simulink model "normal"  (R2023a)
settings: Solver=VariableStepAuto  StartTime=0.0  StopTime=0.2  RelTol=1e-3
libraries: spsMosfetLib x4, spsOnDelayLib x4, spsCurrentMeasurementLib x1, spsDCVoltageSourceLib x1, spsSeriesRLCLoadLib x1, spsTriangleGeneratorLib x1, spsVoltageMeasurementLib x1, sps_lib x1
settings Model: Creator=student  LastModifiedBy=student

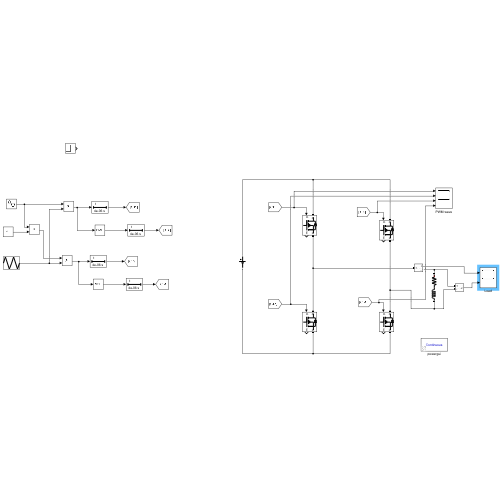
[thumbnail: Simulink's stored preview of the top-level diagram]
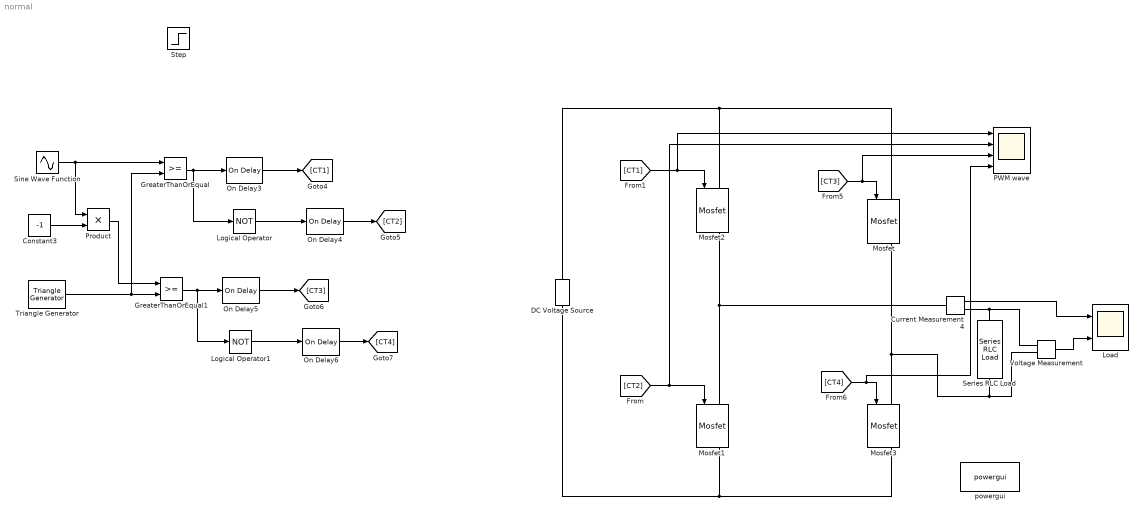
== system normal ==
  Constant3 : Constant  Value=-1
  Current Measurement4 : spsCurrentMeasurementLib/Current Measurement  PhasorSimulation=off  OutputType=Complex  PSBequivalent=0
  DC Voltage Source : spsDCVoltageSourceLib/DC Voltage Source  Amplitude=200  Measurements=None
  GreaterThanOrEqual : RelationalOperator  OutDataTypeStr=boolean  RndMeth=Simplest  InputSameDT=off
  GreaterThanOrEqual1 : RelationalOperator  OutDataTypeStr=boolean  RndMeth=Simplest  InputSameDT=off
  Load : Scope  NumInputPorts=2
  Logical Operator : Logic  Operator=NOT  AllPortsSameDT=off  OutDataTypeStr=boolean
  Logical Operator1 : Logic  Operator=NOT  AllPortsSameDT=off  OutDataTypeStr=boolean
  Mosfet{,1..3} (4 alike) : spsMosfetLib/Mosfet  Ron=0.1  Lon=0  Rd=0.01  Vfd=0  IC=0  Rs=1e5  Cs=inf  Measurements=on
  On Delay{3..6} (4 alike) : spsOnDelayLib/On Delay  DelayType=On delay  delay=4e-06  ic=0  Ts=0
  PWM wave : Scope  NumInputPorts=4
  Product : Product
  Series RLC Load : spsSeriesRLCLoadLib/Series RLC Load  LConnTagsString=a  RConnTagsString=__new0  NominalVoltage=200  NominalFrequency=50  ActivePower=10e3  InductivePower=500  CapacitivePower=0  Setx0=off  InitialVoltage=0  SetiL0=off  InitialCurrent=0  Measurements=None  LoadType=constant Z
  Sine Wave Function : Sin  Amplitude=0.9  Frequency=314.15  SampleTime=0
  Step : Step  Time=0.02  SampleTime=0
  Triangle Generator : spsTriangleGeneratorLib/Triangle Generator  Freq=10000  Phase=90  Ts=0
  Voltage Measurement : spsVoltageMeasurementLib/Voltage Measurement  PhasorSimulation=off  OutputType=Complex  PSBequivalent=0
  powergui : sps_lib/powergui  Priority=1  SimulationMode=Continuous  SampleTime=50e-6  frequency=60  Iterations=50  frequencyindice=0  Pbase=100e6  ErrMax=1e-4  UnitsV=kV  UnitsW=MW  buscounter=0  FunctionMessages=off  echomessages=off  EnableUseOfTLC=off  CurrentSourceSwitches=off  DisableSnubberDevices=off  DisableRonSwitches=off  DisableVfSwitches=off  DisplayEquations=off  AutomaticDiscreteSolvers=off  SolverType=Tustin/Backward Euler (TBE)  Interpol=off  ExternalGateDelay=off  methode=off  Ts=100  x0status=blocks  SPID=on  SwTol=0  HookPort=off  NonlinearTolerance=1e-4  nMaxIteration=100  ContinueOnMaxIteration=off  RestoreLinks=warning  ResistiveCurrentMeasurement=off  Frange=[0:2:500]  Ylog=off  Xlog=on  ShowGrid=off  save=off  variable=ZData  structure=0  ZoomFFT=off  StartTime=0.0  cycles=1  DisplayStyle=1  fundamental=60  FreqAxis=off  MaxFrequency=1000  frequencyindicesteady=1  RmsSteady=1  display=off
  wires:
  [CT4] -> PWM wave/4, Mosfet3/1
  [CT2] -> PWM wave/2, Mosfet1/1
  [CT3] -> PWM wave/3, Mosfet/1
  [CT1] -> PWM wave/1, Mosfet2/1
  Current Measurement4/1 -> Load/1
  Voltage Measurement/1 -> Load/2
  Logical Operator/1 -> On Delay4/1
  Logical Operator1/1 -> On Delay6/1
  GreaterThanOrEqual/1 -> On Delay3/1, Logical Operator/1
  Sine Wave Function/1 -> GreaterThanOrEqual/1, Product/1
  On Delay5/1 -> [CT3]
  Triangle Generator/1 -> GreaterThanOrEqual1/2, GreaterThanOrEqual/2
  Constant3/1 -> Product/2
  On Delay6/1 -> [CT4]
  Product/1 -> GreaterThanOrEqual1/1
  GreaterThanOrEqual1/1 -> On Delay5/1, Logical Operator1/1
  On Delay4/1 -> [CT2]
  On Delay3/1 -> [CT1]
  connections:
  Current Measurement4/RConn1 -- Series RLC Load/LConn1 -- Voltage Measurement/LConn1
  Mosfet2/LConn1 -- DC Voltage Source/RConn1 -- Mosfet/LConn1
  Mosfet2/RConn1 -- Current Measurement4/LConn1 -- Mosfet1/LConn1
  Mosfet/RConn1 -- Series RLC Load/RConn1 -- Voltage Measurement/LConn2 -- Mosfet3/LConn1
  Mosfet3/RConn1 -- DC Voltage Source/LConn1 -- Mosfet1/RConn1
